simulink model "BLDC_Example"  (R2023b)
settings: Solver=ode45  StartTime=0.0  StopTime=10.0  RelTol=1e-3  EnableMultiTasking=on
undefined symbols (not defined in the file): Ts
libraries: simulink x6, spsVoltageMeasurementLib x2, spsDCVoltageSourceLib x1, spsPermanentMagnetSynchronousMachineLib x1, spsUniversalBridgeLib x1, spspowerguiLib x1
settings Model: Creator=hbrsu  LastModifiedBy=84339
settings SolverCC: AlgebraicLoopSolver=TrustRegion
settings DataIOCC: LimitDataPoints=on  SaveFormat=Array  ReturnWorkspaceOutputs=off
settings OptimizationCC: LifeSpan=inf
settings DebuggingCC: UnderspecifiedInitializationDetection=Classic  MergeDetectMultiDrivingBlocksExec=none  SolverPrmCheckMsg=warning  UnconnectedInputMsg=warning  UnconnectedOutputMsg=warning  UnconnectedLineMsg=warning  StateNameClashWarn=warning  SFUnexpectedBacktrackingDiag=warning  SFNoUnconditionalDefaultTransitionDiag=warning  SFExecutionAtInitializationDiag=none  ArithmeticOperatorsInVariantConditions=warning
settings HardwareCC: ProdBitPerPointer=32  ProdBitPerSizeT=32  ProdBitPerPtrDiffT=32  ProdLargestAtomicFloat=None  ProdIntDivRoundTo=Undefined  ProdEndianess=Unspecified  ProdWordSize=32  ProdHWDeviceType=32-bit Generic
settings ModelReferenceCC: PropagateSignalLabelsOutOfModel=off
settings SFSimCC: SimUseLocalCustomCode=off  CustomCodeUndefinedFunction=UseInterfaceOnly
settings RTWCC: RTWUseLocalCustomCode=off
settings CodeAppCC: StateflowObjectComments=on
settings GRTTargetCC: TargetLangStandard=C89/C90 (ANSI)
settings ConfigComp: CovMetricSettings=dw  CovSaveCumulativeToWorkspaceVar=on  CovSaveSingleToWorkspaceVar=on  CovExternalEMLEnable=off
settings SimscapeCC: SimscapeNormalizeSystem=off

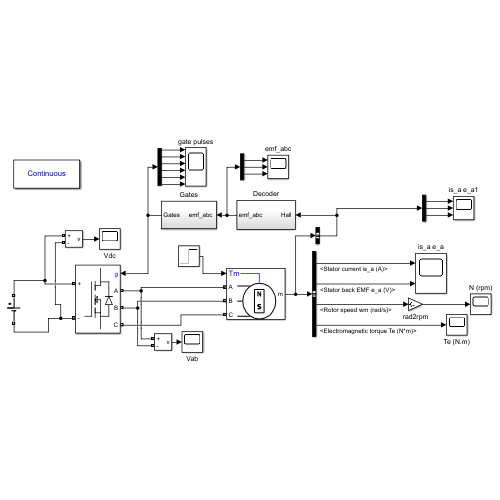
[thumbnail: Simulink's stored preview of the top-level diagram]
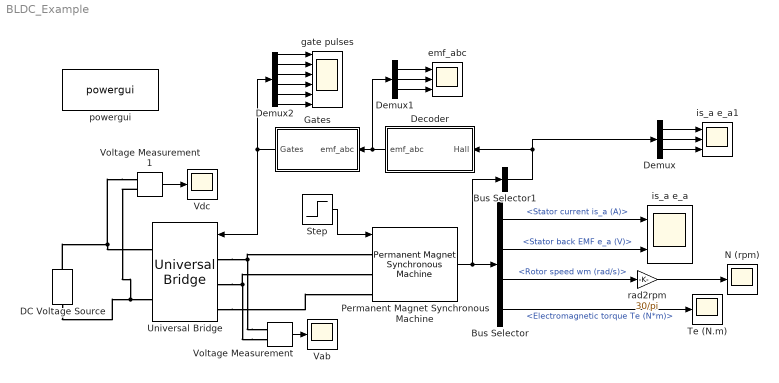
== system BLDC_Example ==
  Bus Selector : BusSelector  OutputSignals=Stator current is_a (A),Stator back EMF e_a (V),Rotor speed wm (rad/s),Electromagnetic torque Te (N*m)
  Bus Selector1 : BusSelector  OutputSignals=Hall effect signal h_a,Hall effect signal h_b,Hall effect signal h_c  OutputAsBus=on
  DC Voltage Source : spsDCVoltageSourceLib/DC Voltage Source  Amplitude=300  Measurements=None
  Decoder : Subsystem
  Demux : Demux  Outputs=3
  Demux1 : Demux  Outputs=3
  Demux2 : Demux  Outputs=6
  Gates : Subsystem
  N (rpm) : Scope
  Permanent Magnet Synchronous Machine : spsPermanentMagnetSynchronousMachineLib/Permanent Magnet Synchronous Machine  NbPhases=3  FluxDistribution=Trapezoidal  RotorType=Round  MechanicalLoad=Torque Tm  PresetModel=No  ShowDetailedParameters=on  MeasurementBus=off  Resistance=2.8750  Inductance=8.5e-3  dqInductances=[8.5e-3, 8.5e-3]  La=0.000835  MachineConstant=Flux linkage established by magnets (V.s)  Flux=0.175  VoltageCst=146.6077  TorqueCst=1.4  Flat=120  Mechanical=[ 0.8e-3, 1e-3 4]  PolePairs=4  InitialConditions=[0,0, 0,0]  InitialConditions5ph=[0 0 0 0 0 0]  RefAngle=90 degrees behind phase A axis (modified Park)  IterativeDiscreteModel=Trapezoidal non iterative  TsBlock=-1  TsPowergui=0
  Step : Step  Time=.1  After=3  SampleTime=0
  Te (N.m) : Scope
  Universal Bridge : spsUniversalBridgeLib/Universal Bridge  Arms=3  SnubberResistance=5000  SnubberCapacitance=1e-6  Device=MOSFET / Diodes  Ron=1e-3  Lon=0  ForwardVoltages="[  0  0  ]"  ForwardVoltage=0  GTOparameters=[ 10e-6 , 20e-6 ]  IGBTparameters=[ 1e-6 , 2e-6 ]  Measurements=None  Measurements_2=None  converterType=Rectifier
  Vab : Scope
  Vdc : Scope
  Voltage Measurement : spsVoltageMeasurementLib/Voltage Measurement  PhasorSimulation=off  OutputType=Complex  PSBequivalent=0
  Voltage Measurement1 : spsVoltageMeasurementLib/Voltage Measurement  PhasorSimulation=off  OutputType=Complex  PSBequivalent=0
  emf_abc : Scope  NumInputPorts=3
  gate pulses : Scope  NumInputPorts=6
  is_a e_a : Scope  NumInputPorts=2
  is_a e_a1 : Scope  NumInputPorts=3
  powergui : spspowerguiLib/powergui  Priority=2  SimulationMode=Continuous  SampleTime=Ts  frequency=60  Iterations=50  frequencyindice=0  Pbase=100e6  ErrMax=1e-4  UnitsV=kV  UnitsW=MW  buscounter=0  FunctionMessages=off  echomessages=off  EnableUseOfTLC=off  CurrentSourceSwitches=on  DisableSnubberDevices=off  DisableRonSwitches=off  DisableVfSwitches=off  DisplayEquations=off  AutomaticDiscreteSolvers=off  SolverType=Tustin  Interpol=off  ExternalGateDelay=off  methode=off  Ts=0  x0status=blocks  SPID=off  SwTol=0  HookPort=off  NonlinearTolerance=1e-4  nMaxIteration=100  ContinueOnMaxIteration=off  RestoreLinks=warning  ResistiveCurrentMeasurement=off  Frange=[0:2:500]  Ylog=off  Xlog=on  ShowGrid=off  save=off  variable=ZData  structure=0  ZoomFFT=on  StartTime=0.0  cycles=1  DisplayStyle=1  fundamental=60  FreqAxis=off  MaxFrequency=1000  frequencyindicesteady=1  RmsSteady=1  display=off
  rad2rpm : Gain  Gain=30/pi
  wires:
  Step/1 -> Permanent Magnet Synchronous Machine/1
  Decoder/1(emf_abc) -> Demux1/1, Gates/1("emf_abc ")
  rad2rpm/1 -> N (rpm)/1
  Voltage Measurement/1 -> Vab/1
  Voltage Measurement1/1 -> Vdc/1
  Bus Selector/1 -> is_a e_a/1  "<Stator current is_a (A)>"
  Permanent Magnet Synchronous Machine/1 -> Bus Selector/1, Bus Selector1/1
  Bus Selector1/1 -> Decoder/1("Hall "), Demux/1
  Bus Selector/2 -> is_a e_a/2  "<Stator back EMF e_a (V)>"
  Bus Selector/3 -> rad2rpm/1  "<Rotor speed wm (rad/s)>"
  Bus Selector/4 -> Te (N.m)/1  "<Electromagnetic torque Te (N*m)>"
  Demux/1 -> is_a e_a1/1
  Demux/2 -> is_a e_a1/2
  Demux/3 -> is_a e_a1/3
  Demux1/1 -> emf_abc/1
  Demux1/2 -> emf_abc/2
  Demux1/3 -> emf_abc/3
  Gates/1(Gates) -> Demux2/1, Universal Bridge/1
  Demux2/1 -> gate pulses/1
  Demux2/2 -> gate pulses/2
  Demux2/3 -> gate pulses/3
  Demux2/4 -> gate pulses/4
  Demux2/5 -> gate pulses/5
  Demux2/6 -> gate pulses/6
  connections:
  Voltage Measurement/LConn1 -- Permanent Magnet Synchronous Machine/LConn1 -- Universal Bridge/LConn1
  Voltage Measurement/LConn2 -- Permanent Magnet Synchronous Machine/LConn2 -- Universal Bridge/LConn2
  Voltage Measurement1/LConn1 -- DC Voltage Source/RConn1 -- Universal Bridge/RConn1
  Universal Bridge/LConn3 -- Permanent Magnet Synchronous Machine/LConn3
  DC Voltage Source/LConn1 -- Voltage Measurement1/LConn2 -- Universal Bridge/RConn2

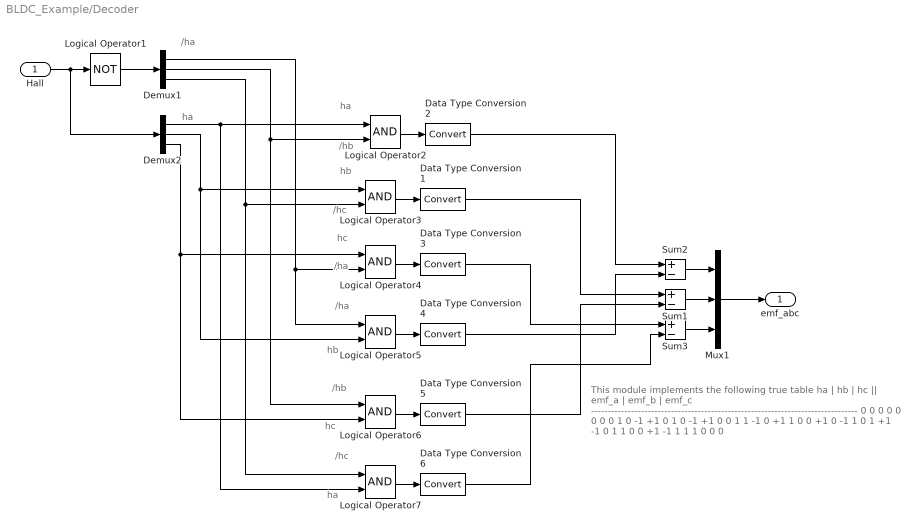
== system BLDC_Example/Decoder ==
  note: /ha
  note: ha
  note: ha
  note: /hb
  note: hb
  note: /hc
  note: hc
  note: /ha
  note: /ha
  note: hb
  note: /hb
  note: hc
  note: /hc
  note: ha
  note: This module implements the following true table
      |
      |    ha   |   hb   |   hc   ||   emf_a   |   emf_b   |   emf_c
      |     --------------------------------------------------------------------------------
      | 0          0         0          0               0               0
      | 0          0         1          0               -1              +1
      | 0          1         0          -1              +1                0
      | 0          1         1          -1               0               +1
      | 1          0         0         +1               0               -1
      | 1          0         1         +1              -1                0
      | 1          1         0          0              +1               -1
      | 1          1         1          0               0                0
  "Hall " : Inport
  Data Type Conversion{1..6} (6 alike) : DataTypeConversion  SaturateOnIntegerOverflow=off  RndMeth=Floor
  Demux1 : Demux  Outputs=3
  Demux2 : Demux  Outputs=3
  Logical Operator1 : Logic  Operator=NOT  AllPortsSameDT=off  OutDataTypeStr=boolean
  Logical Operator{2..7} (6 alike) : Logic  AllPortsSameDT=off  OutDataTypeStr=boolean
  Mux1 : Mux  Inputs=3
  Sum1 : Sum  Inputs=+-  OutDataTypeStr=double
  Sum2 : Sum  Inputs=+-  OutDataTypeStr=double
  Sum3 : Sum  Inputs=+-  OutDataTypeStr=double
  emf_abc : Outport
  wires:
  "Hall "/1 -> Logical Operator1/1, Demux2/1
  Logical Operator1/1 -> Demux1/1
  Demux2/3 -> Logical Operator4/1, Logical Operator6/2
  Demux2/2 -> Logical Operator3/1, Logical Operator5/2
  Demux2/1 -> Logical Operator2/1, Logical Operator7/2
  Demux1/3 -> Logical Operator3/2, Logical Operator7/1
  Demux1/2 -> Logical Operator2/2, Logical Operator6/1
  Demux1/1 -> Logical Operator4/2, Logical Operator5/1
  Logical Operator2/1 -> Data Type Conversion2/1
  Sum2/1 -> Mux1/1
  Sum1/1 -> Mux1/2
  Sum3/1 -> Mux1/3
  Mux1/1 -> emf_abc/1
  Logical Operator3/1 -> Data Type Conversion1/1
  Logical Operator4/1 -> Data Type Conversion3/1
  Logical Operator5/1 -> Data Type Conversion4/1
  Logical Operator6/1 -> Data Type Conversion5/1
  Logical Operator7/1 -> Data Type Conversion6/1
  Data Type Conversion2/1 -> Sum2/1
  Data Type Conversion4/1 -> Sum2/2
  Data Type Conversion1/1 -> Sum1/1
  Data Type Conversion5/1 -> Sum1/2
  Data Type Conversion3/1 -> Sum3/1
  Data Type Conversion6/1 -> Sum3/2

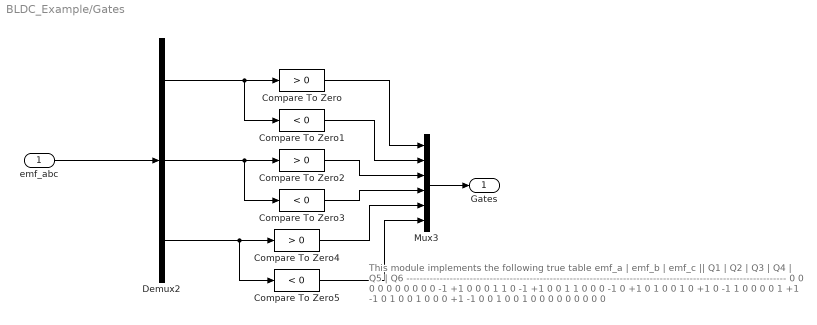
== system BLDC_Example/Gates ==
  note: This module implements the following true table
      |
      |    emf_a   |   emf_b   |   emf_c   ||   Q1   |   Q2   |   Q3   |   Q4   |   Q5   |   Q6
      |     ------------------------------------------------------------------------------------------------------------------
      |       0              0                0            0          0          0           0        0        0
      |       0               -1              +1          0          0          0           1        1        0
      |     -1              +1                0          0          1          1           0        0        0
      |     -1               0               +1          0          1         0           0        1        0
      |    +1               0                -1          1          0          0           0        0        1
      |    +1              -1                0           1          0          0           1        0        0
      |      0              +1               -1           0          0          1           0        0        1
      |     0              0                0             0          0          0           0        0        0
  "emf_abc " : Inport
  Compare To Zero : simulink/Logic and Bit Operations/Compare To Zero  relop=>  OutDataTypeStr=boolean  ZeroCross=off
  Compare To Zero1 : simulink/Logic and Bit Operations/Compare To Zero  relop=<  OutDataTypeStr=boolean  ZeroCross=off
  Compare To Zero2 : simulink/Logic and Bit Operations/Compare To Zero  relop=>  OutDataTypeStr=boolean  ZeroCross=off
  Compare To Zero3 : simulink/Logic and Bit Operations/Compare To Zero  relop=<  OutDataTypeStr=boolean  ZeroCross=off
  Compare To Zero4 : simulink/Logic and Bit Operations/Compare To Zero  relop=>  OutDataTypeStr=boolean  ZeroCross=off
  Compare To Zero5 : simulink/Logic and Bit Operations/Compare To Zero  relop=<  OutDataTypeStr=boolean  ZeroCross=off
  Demux2 : Demux  Outputs=3
  Mux3 : Mux  Inputs=6
  Gates : Outport
  wires:
  "emf_abc "/1 -> Demux2/1
  Mux3/1 -> Gates/1
  Demux2/1 -> Compare To Zero/1, Compare To Zero1/1
  Demux2/2 -> Compare To Zero2/1, Compare To Zero3/1
  Demux2/3 -> Compare To Zero4/1, Compare To Zero5/1
  Compare To Zero/1 -> Mux3/1
  Compare To Zero1/1 -> Mux3/2
  Compare To Zero2/1 -> Mux3/3
  Compare To Zero3/1 -> Mux3/4
  Compare To Zero4/1 -> Mux3/5
  Compare To Zero5/1 -> Mux3/6
